simulink model "PID"  (R2025a)
settings: Solver=FixedStepAuto  StartTime=0.0  StopTime=50  FixedStep=0.001  RelTol=1e-3
values from neighbouring files (symbols this model uses):
  g = 9.81    [param.m]
  Iv = diag([1e-2, 8.2e-3, 1.48e-2])    [param.m]
  kd = 0.0487    [param.m]
  Kd_att = [0 0 0]'    [param.m]
  Kd_att_dot = [0.0006 0.0004 0.0]'    [param.m]
  Kd_vel = [0.2 0.2 0]'    [param.m]
  Ki_att = [0 0 0]'    [param.m]
  Ki_att_dot = [0.1 0.1 0.1]'    [param.m]
  Ki_vel = [0.4 0.4 2.0]'    [param.m]
  Kp_att = [6.5 6.5 0.4]'    [param.m]
  Kp_att_dot = [0.053 0.055 0.09]'    [param.m]
  Kp_pos = [0.5 0.5 1]'    [param.m]
  Kp_vel = [1.8 1.8 4]'    [param.m]
  kt = 5.11    [param.m]
  Lpitch = 0.1758    [param.m]
  Lroll = 0.2136    [param.m]
  m = 1.121    [param.m]
settings Model: Creator=huy01  LastModifiedBy=huy01
settings SolverCC: ZeroCrossAlgorithm=Adaptive
settings DebuggingCC: IgnoredZcDiagnostic=none

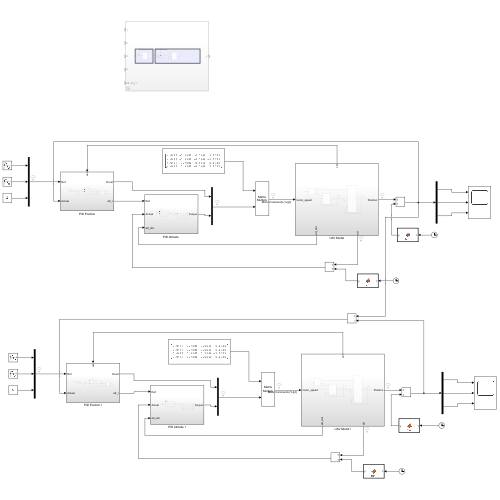
[thumbnail: Simulink's stored preview of the top-level diagram]
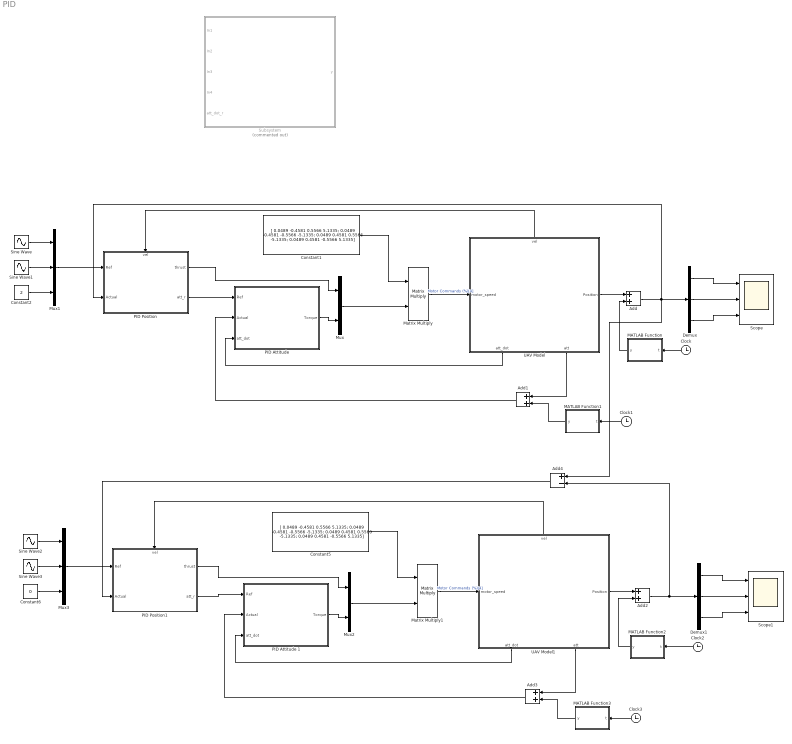
== system PID ==
  Add{,1..3} (4 alike) : Sum
  Add4 : Sum  Inputs=+-
  Clock{,1..3} (4 alike) : Clock
  Constant1 : Constant  Value=|
      | [ 0.0489   -0.4581    0.5566    5.1335;
      |   0.0489   -0.4581   -0.5566   -5.1335;
      |   0.0489    0.4581    0.5566   -5.1335;
      |   0.0489    0.4581   -0.5566    5.1335]
  Constant2 : Constant  Value=2
  Constant5 : Constant  Value=|
      | [ 0.0489   -0.4581    0.5566    5.1335;
      |   0.0489   -0.4581   -0.5566   -5.1335;
      |   0.0489    0.4581    0.5566   -5.1335;
      |   0.0489    0.4581   -0.5566    5.1335]
  Constant6 : Constant  Value=0
  Demux : Demux  Outputs=3
  Demux1 : Demux  Outputs=3
  MATLAB Function : MATLAB Function  TreatAsAtomicUnit=on
  MATLAB Function1 : MATLAB Function  TreatAsAtomicUnit=on
  MATLAB Function2 : MATLAB Function  TreatAsAtomicUnit=on
  MATLAB Function3 : MATLAB Function  TreatAsAtomicUnit=on
  Matrix Multiply : Product  Multiplication=Matrix(*)
  Matrix Multiply1 : Product  Multiplication=Matrix(*)
  Mux : Mux  Inputs=2
  Mux1 : Mux  Inputs=3
  Mux2 : Mux  Inputs=2
  Mux3 : Mux  Inputs=3
  "PID Attitude " : Subsystem
  PID Attitude 1 : Subsystem
  PID Position : Subsystem
      settings: PortSchema="{\"entries\":[{\"content\":{\"sides\":[{\"content\":{\"connectorIds\":[\"In1\",\"In2\"]},\"type\":\"ConnectorPlacement.EquallySpacedRectSide\",\"uuid\":\"8ef4bc25-06d7-445e-a37a-ff1ebe3f11af\"},{\"content\":{\"connectorIds\":[\"Out1\",\"Out2\"],\"side\":\"RIGHT\"},\"type\":\"ConnectorPlacement.EquallySpacedRectSide\",\"uuid\":\"499381c3-f9a0-4f2e-8347-7eacec8f48af\"},{\"content\":{\"connectorIds\":[\"In3\"],\"side\":\"TOP\"},\"type\":\"ConnectorPlacement.EquallySpacedRectSide\",\"uuid\":\"0d907384-0ff5-4165-8e8f-a88dac793d14\"}]},\"type\":\"ConnectorPlacement.EquallySpacedConnector\",\"uuid\":\"f2c7b912-1bff-4caa-903e-36b65c99468e\"}],\"packageUris\":[\"http://schema.mathworks.com/mf0/Connector/R2020b\"],\"version\":\"1.0\"}"
  PID Position1 : Subsystem
      settings: PortSchema="{\"entries\":[{\"content\":{\"sides\":[{\"content\":{\"connectorIds\":[\"In1\",\"In2\"]},\"type\":\"ConnectorPlacement.EquallySpacedRectSide\",\"uuid\":\"757670a2-abb9-46b8-b8ef-ade2779e4005\"},{\"content\":{\"connectorIds\":[\"Out1\",\"Out2\"],\"side\":\"RIGHT\"},\"type\":\"ConnectorPlacement.EquallySpacedRectSide\",\"uuid\":\"80a4837c-f927-466b-93fb-175090a45c5c\"},{\"content\":{\"connectorIds\":[\"In3\"],\"side\":\"TOP\"},\"type\":\"ConnectorPlacement.EquallySpacedRectSide\",\"uuid\":\"6659d1df-ad98-411a-9518-a7cd5dbf3d7b\"}]},\"type\":\"ConnectorPlacement.EquallySpacedConnector\",\"uuid\":\"7846e0cb-a6a7-4697-994f-28587a096689\"}],\"packageUris\":[\"http://schema.mathworks.com/mf0/Connector/R2020b\"],\"version\":\"1.0\"}"
  Scope : Scope  NumInputPorts=3
      settings: ActiveDisplayYMinimum=-0.13419918718369481  ActiveDisplayYMaximum=1.1736814894873611  DataLoggingVariableName=ScopeData2
  Scope1 : Scope  NumInputPorts=3
      settings: ActiveDisplayYMinimum=-2.707243758032325  ActiveDisplayYMaximum=2.7233489767493806  DataLoggingVariableName=ScopeData3
  Sine Wave : Sin  Amplitude=2  Frequency=pi/18  SampleTime=0
  Sine Wave1 : Sin  Amplitude=2  Frequency=pi/18  Phase=pi/2  SampleTime=0
  Sine Wave2 : Sin  Amplitude=4  Frequency=pi/18  SampleTime=0
  Sine Wave3 : Sin  Amplitude=4  Frequency=pi/18  Phase=pi/2  SampleTime=0
  Subsystem : Subsystem  Commented=on
  UAV Model : Subsystem
      settings: PortSchema="{\"entries\":[{\"content\":{\"sides\":[{\"content\":{\"connectorIds\":[\"In1\"]},\"type\":\"ConnectorPlacement.EquallySpacedRectSide\",\"uuid\":\"e9a53653-5fbc-46c1-971d-b6f83c711259\"},{\"content\":{\"connectorIds\":[\"Out1\"],\"side\":\"RIGHT\"},\"type\":\"ConnectorPlacement.EquallySpacedRectSide\",\"uuid\":\"e2104fa5-1b8a-4227-a89f-dda87c76df89\"},{\"content\":{\"connectorIds\":[\"Out4\"],\"side\":\"TOP\"},\"type\":\"ConnectorPlacement.EquallySpacedRectSide\",\"uuid\":\"f4bec026-a14b-467a-8c55-ded87294653f\"},{\"content\":{\"connectorIds\":[\"Out2\",\"Out3\"],\"side\":\"BOTTOM\"},\"type\":\"ConnectorPlacement.EquallySpacedRectSide\",\"uuid\":\"97e6d9ca-da58-485e-9073-412d9dc474d6\"}]},\"type\":\"ConnectorPlacement.EquallySpacedConnector\",\"uuid\":\"03146a94-fd08-496a-b759-aae2d503529b\"}],\"packageUris\":[\"http://schema.mathworks.com/mf0/Connector/R2020b\"],\"version\":\"1.0\"}"
  UAV Model1 : Subsystem
      settings: PortSchema="{\"entries\":[{\"content\":{\"sides\":[{\"content\":{\"connectorIds\":[\"In1\"]},\"type\":\"ConnectorPlacement.EquallySpacedRectSide\",\"uuid\":\"e9a53653-5fbc-46c1-971d-b6f83c711259\"},{\"content\":{\"connectorIds\":[\"Out1\"],\"side\":\"RIGHT\"},\"type\":\"ConnectorPlacement.EquallySpacedRectSide\",\"uuid\":\"e2104fa5-1b8a-4227-a89f-dda87c76df89\"},{\"content\":{\"connectorIds\":[\"Out4\"],\"side\":\"TOP\"},\"type\":\"ConnectorPlacement.EquallySpacedRectSide\",\"uuid\":\"f4bec026-a14b-467a-8c55-ded87294653f\"},{\"content\":{\"connectorIds\":[\"Out2\",\"Out3\"],\"side\":\"BOTTOM\"},\"type\":\"ConnectorPlacement.EquallySpacedRectSide\",\"uuid\":\"97e6d9ca-da58-485e-9073-412d9dc474d6\"}]},\"type\":\"ConnectorPlacement.EquallySpacedConnector\",\"uuid\":\"03146a94-fd08-496a-b759-aae2d503529b\"}],\"packageUris\":[\"http://schema.mathworks.com/mf0/Connector/R2020b\"],\"version\":\"1.0\"}"
  wires:
  PID Position/2(att_r) -> "PID Attitude "/1("Ref ")
  UAV Model/2(att_dot) -> "PID Attitude "/3(att_dot)
  "PID Attitude "/1(Torque) -> Mux/2
  PID Position/1(thrust) -> Mux/1
  Mux/1 -> Matrix Multiply/2
  Constant1/1 -> Matrix Multiply/1
  Mux1/1 -> PID Position/1("Ref ")
  Demux/1 -> Scope/1
  Demux/2 -> Scope/2
  Demux/3 -> Scope/3
  Constant2/1 -> Mux1/3
  Sine Wave/1 -> Mux1/1
  Sine Wave1/1 -> Mux1/2
  MATLAB Function/1(y) -> Add/2
  Clock/1 -> MATLAB Function/1(t)
  UAV Model/1(Position) -> Add/1
  Add/1 -> Add4/1, PID Position/2(Actual), Demux/1
  UAV Model/3(att) -> Add1/1
  Add1/1 -> "PID Attitude "/2(Actual)
  MATLAB Function1/1(y) -> Add1/2
  Clock1/1 -> MATLAB Function1/1(t)
  Matrix Multiply/1 -> UAV Model/1(motor_speed)  "Motor Commands (%)[4]"
  Matrix Multiply1/1 -> UAV Model1/1(motor_speed)  "Motor Commands (%)[4]"
  UAV Model1/1(Position) -> Add2/1
  MATLAB Function2/1(y) -> Add2/2
  MATLAB Function3/1(y) -> Add3/2
  Clock2/1 -> MATLAB Function2/1(t)
  UAV Model1/3(att) -> Add3/1
  Constant6/1 -> Mux3/3
  Sine Wave2/1 -> Mux3/1
  Demux1/3 -> Scope1/3
  PID Position1/2(att_r) -> PID Attitude 1/1("Ref ")
  Constant5/1 -> Matrix Multiply1/1
  Clock3/1 -> MATLAB Function3/1(t)
  Add2/1 -> Demux1/1, Add4/2
  PID Position1/1(thrust) -> Mux2/1
  Mux2/1 -> Matrix Multiply1/2
  UAV Model1/2(att_dot) -> PID Attitude 1/3(att_dot)
  Mux3/1 -> PID Position1/1("Ref ")
  Add3/1 -> PID Attitude 1/2(Actual)
  Demux1/2 -> Scope1/2
  Sine Wave3/1 -> Mux3/2
  PID Attitude 1/1(Torque) -> Mux2/2
  Demux1/1 -> Scope1/1
  Add4/1 -> PID Position1/2(Actual)
  UAV Model/4(vel) -> PID Position/3(vel)
  UAV Model1/4(vel) -> PID Position1/3(vel)

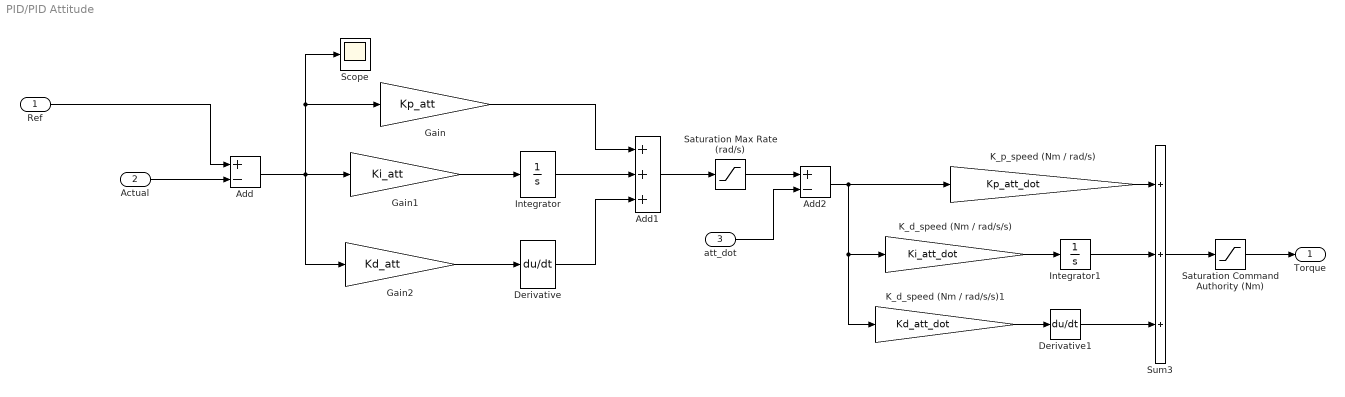
== system PID/PID Attitude  ==
  "Ref " : Inport
  Actual : Inport  Port=2
  att_dot : Inport  Port=3
  Add : Sum  Inputs=+-
  Add1 : Sum  Inputs=+++
  Add2 : Sum  Inputs=+-
  Derivative : Derivative
  Derivative1 : Derivative
  Gain : Gain  Gain=Kp_att
  Gain1 : Gain  Gain=Ki_att
  Gain2 : Gain  Gain=Kd_att
  Integrator : Integrator
  Integrator1 : Integrator
  K_d_speed (Nm / rad/s/s) : Gain  Gain=Ki_att_dot
  K_d_speed (Nm / rad/s/s)1 : Gain  Gain=Kd_att_dot
  K_p_speed (Nm / rad/s) : Gain  Gain=Kp_att_dot
  Saturation Command Authority (Nm) : Saturate  UpperLimit=[1.0915 0.8984 0.0984]'  LowerLimit=-[1.0915 0.8984 0.0984]'
  Saturation Max Rate (rad/s) : Saturate  UpperLimit=10*pi/3*[1 1 1]'  LowerLimit=-10*pi/3*[1 1 1]'
  Scope : Scope
      settings: ActiveDisplayYMinimum=-1  ActiveDisplayYMaximum=1  DataLoggingVariableName=ScopeData5
  Sum3 : Sum  Inputs=+++
  Torque : Outport
  wires:
  Actual/1 -> Add/2
  Add/1 -> Gain2/1, Gain1/1, Gain/1, Scope/1
  Gain1/1 -> Integrator/1
  Integrator/1 -> Add1/2
  Gain/1 -> Add1/1
  Gain2/1 -> Derivative/1
  Derivative/1 -> Add1/3
  "Ref "/1 -> Add/1
  Add1/1 -> Saturation Max Rate (rad/s)/1
  K_d_speed (Nm / rad/s/s)/1 -> Integrator1/1
  K_p_speed (Nm / rad/s)/1 -> Sum3/1
  Saturation Max Rate (rad/s)/1 -> Add2/1
  att_dot/1 -> Add2/2
  Integrator1/1 -> Sum3/2
  K_d_speed (Nm / rad/s/s)1/1 -> Derivative1/1
  Derivative1/1 -> Sum3/3
  Add2/1 -> K_d_speed (Nm / rad/s/s)1/1, K_d_speed (Nm / rad/s/s)/1, K_p_speed (Nm / rad/s)/1
  Sum3/1 -> Saturation Command Authority (Nm)/1
  Saturation Command Authority (Nm)/1 -> Torque/1

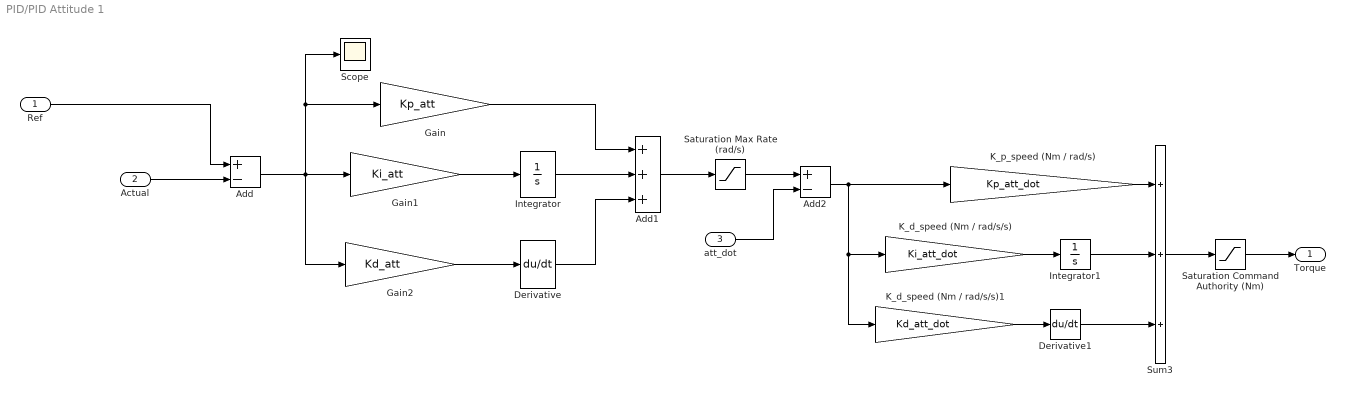
== system PID/PID Attitude 1 ==
  "Ref " : Inport
  Actual : Inport  Port=2
  att_dot : Inport  Port=3
  Add : Sum  Inputs=+-
  Add1 : Sum  Inputs=+++
  Add2 : Sum  Inputs=+-
  Derivative : Derivative
  Derivative1 : Derivative
  Gain : Gain  Gain=Kp_att
  Gain1 : Gain  Gain=Ki_att
  Gain2 : Gain  Gain=Kd_att
  Integrator : Integrator
  Integrator1 : Integrator
  K_d_speed (Nm / rad/s/s) : Gain  Gain=Ki_att_dot
  K_d_speed (Nm / rad/s/s)1 : Gain  Gain=Kd_att_dot
  K_p_speed (Nm / rad/s) : Gain  Gain=Kp_att_dot
  Saturation Command Authority (Nm) : Saturate  UpperLimit=[1.0915 0.8984 0.0984]'  LowerLimit=-[1.0915 0.8984 0.0984]'
  Saturation Max Rate (rad/s) : Saturate  UpperLimit=10*pi/3*[1 1 1]'  LowerLimit=-10*pi/3*[1 1 1]'
  Scope : Scope
      settings: ActiveDisplayYMinimum=-1  ActiveDisplayYMaximum=1  DataLoggingVariableName=ScopeData5
  Sum3 : Sum  Inputs=+++
  Torque : Outport
  wires:
  Actual/1 -> Add/2
  Add/1 -> Gain2/1, Gain1/1, Gain/1, Scope/1
  Gain1/1 -> Integrator/1
  Integrator/1 -> Add1/2
  Gain/1 -> Add1/1
  Gain2/1 -> Derivative/1
  Derivative/1 -> Add1/3
  "Ref "/1 -> Add/1
  Add1/1 -> Saturation Max Rate (rad/s)/1
  K_d_speed (Nm / rad/s/s)/1 -> Integrator1/1
  K_p_speed (Nm / rad/s)/1 -> Sum3/1
  Saturation Max Rate (rad/s)/1 -> Add2/1
  att_dot/1 -> Add2/2
  Integrator1/1 -> Sum3/2
  K_d_speed (Nm / rad/s/s)1/1 -> Derivative1/1
  Derivative1/1 -> Sum3/3
  Add2/1 -> K_d_speed (Nm / rad/s/s)1/1, K_d_speed (Nm / rad/s/s)/1, K_p_speed (Nm / rad/s)/1
  Sum3/1 -> Saturation Command Authority (Nm)/1
  Saturation Command Authority (Nm)/1 -> Torque/1

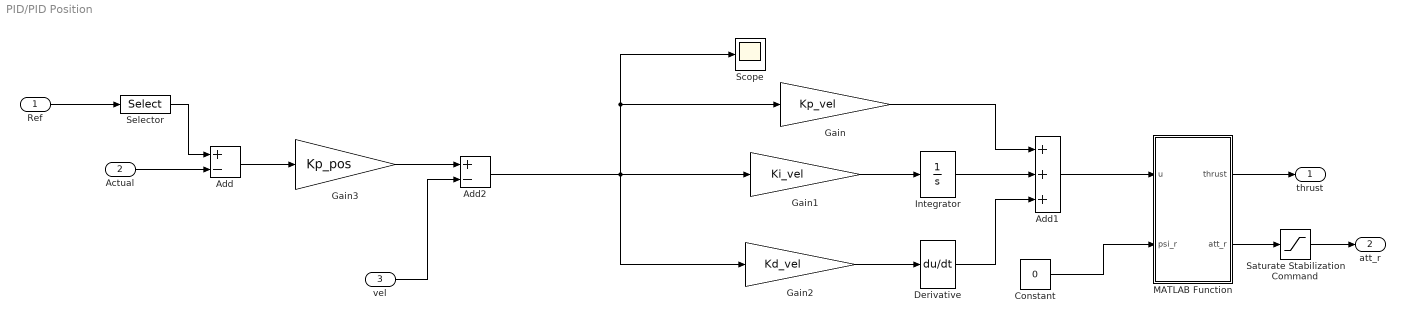
== system PID/PID Position ==
  "Ref " : Inport
  Actual : Inport  Port=2
  vel : Inport  Port=3
  Add : Sum  Inputs=+-
  Add1 : Sum  Inputs=+++
  Add2 : Sum  Inputs=+-
  Constant : Constant  Value=0
  Derivative : Derivative
  Gain : Gain  Gain=Kp_vel
  Gain1 : Gain  Gain=Ki_vel
  Gain2 : Gain  Gain=Kd_vel
  Gain3 : Gain  Gain=Kp_pos
  Integrator : Integrator
  MATLAB Function : MATLAB Function  TreatAsAtomicUnit=on  mask{m=m, g=g}
      mask prompts: m "Mass"; g "Gravity"
  Saturate Stabilization Command : Saturate  UpperLimit=[pi/4 pi/4 inf]'  LowerLimit=[-pi/4 -pi/4 -inf]'
  Scope : Scope
      settings: ActiveDisplayYMinimum=-3.266677596790764  ActiveDisplayYMaximum=4.2877709714359939  DataLoggingVariableName=ScopeData4
  Selector : Selector  InputPortWidth=3  IndexOptions=Index vector (dialog)  Indices=[1:3]  OutputSizes=1
  thrust : Outport
  att_r : Outport  Port=2
  wires:
  Actual/1 -> Add/2
  Gain1/1 -> Integrator/1
  Integrator/1 -> Add1/2
  Gain/1 -> Add1/1
  Gain2/1 -> Derivative/1
  Derivative/1 -> Add1/3
  Add1/1 -> MATLAB Function/1(u)
  "Ref "/1 -> Selector/1
  Selector/1 -> Add/1
  MATLAB Function/1(thrust) -> thrust/1
  MATLAB Function/2(att_r) -> Saturate Stabilization Command/1
  Saturate Stabilization Command/1 -> att_r/1
  Constant/1 -> MATLAB Function/2(psi_r)
  Add/1 -> Gain3/1
  Gain3/1 -> Add2/1
  Add2/1 -> Gain2/1, Gain1/1, Gain/1, Scope/1
  vel/1 -> Add2/2

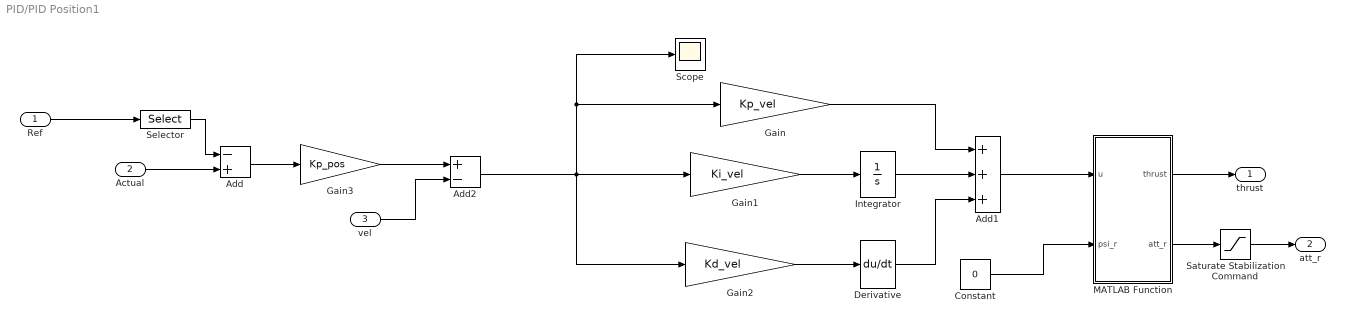
== system PID/PID Position1 ==
  "Ref " : Inport
  Actual : Inport  Port=2
  vel : Inport  Port=3
  Add : Sum  Inputs=-+
  Add1 : Sum  Inputs=+++
  Add2 : Sum  Inputs=+-
  Constant : Constant  Value=0
  Derivative : Derivative
  Gain : Gain  Gain=Kp_vel
  Gain1 : Gain  Gain=Ki_vel
  Gain2 : Gain  Gain=Kd_vel
  Gain3 : Gain  Gain=Kp_pos
  Integrator : Integrator
  MATLAB Function : MATLAB Function  TreatAsAtomicUnit=on  mask{m=m, g=g}
      mask prompts: m "Mass"; g "Gravity"
  Saturate Stabilization Command : Saturate  UpperLimit=[pi/4 pi/4 inf]'  LowerLimit=[-pi/4 -pi/4 -inf]'
  Scope : Scope
      settings: ActiveDisplayYMinimum=-3.266677596790764  ActiveDisplayYMaximum=4.2877709714359939  DataLoggingVariableName=ScopeData4
  Selector : Selector  InputPortWidth=3  IndexOptions=Index vector (dialog)  Indices=[1:3]  OutputSizes=1
  thrust : Outport
  att_r : Outport  Port=2
  wires:
  Actual/1 -> Add/2
  Gain1/1 -> Integrator/1
  Integrator/1 -> Add1/2
  Gain/1 -> Add1/1
  Gain2/1 -> Derivative/1
  Derivative/1 -> Add1/3
  Add1/1 -> MATLAB Function/1(u)
  "Ref "/1 -> Selector/1
  Selector/1 -> Add/1
  MATLAB Function/1(thrust) -> thrust/1
  MATLAB Function/2(att_r) -> Saturate Stabilization Command/1
  Saturate Stabilization Command/1 -> att_r/1
  Constant/1 -> MATLAB Function/2(psi_r)
  Add/1 -> Gain3/1
  Gain3/1 -> Add2/1
  Add2/1 -> Gain2/1, Scope/1, Gain/1, Gain1/1
  vel/1 -> Add2/2

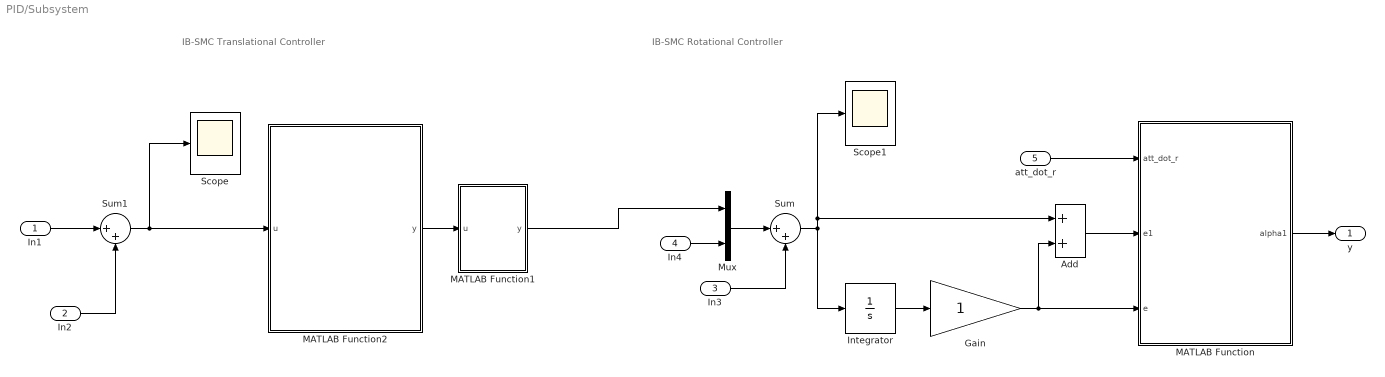
== system PID/Subsystem ==
  note: IB-SMC Translational Controller
  note: IB-SMC Rotational Controller
  In1 : Inport
  In2 : Inport  Port=2
  In3 : Inport  Port=3
  In4 : Inport  Port=4
  att_dot_r : Inport  Port=5
  Add : Sum
  Gain : Gain
  Integrator : Integrator
  MATLAB Function : MATLAB Function  TreatAsAtomicUnit=on
  MATLAB Function1 : MATLAB Function  TreatAsAtomicUnit=on
  MATLAB Function2 : MATLAB Function  TreatAsAtomicUnit=on
  Mux : Mux  Inputs=2
  Scope : Scope
  Scope1 : Scope
  Sum : Sum  Inputs=|++
  Sum1 : Sum  Inputs=|++
  y : Outport
  wires:
  Sum1/1 -> Scope/1, MATLAB Function2/1(u)
  In3/1 -> Sum/2
  MATLAB Function/1(alpha1) -> y/1
  Sum/1 -> Scope1/1, Add/1, Integrator/1
  MATLAB Function2/1(y) -> MATLAB Function1/1(u)
  In2/1 -> Sum1/2
  In1/1 -> Sum1/1
  Mux/1 -> Sum/1
  MATLAB Function1/1(y) -> Mux/1
  In4/1 -> Mux/2
  Integrator/1 -> Gain/1
  Gain/1 -> Add/2, MATLAB Function/3(e)
  Add/1 -> MATLAB Function/2(e1)
  att_dot_r/1 -> MATLAB Function/1(att_dot_r)

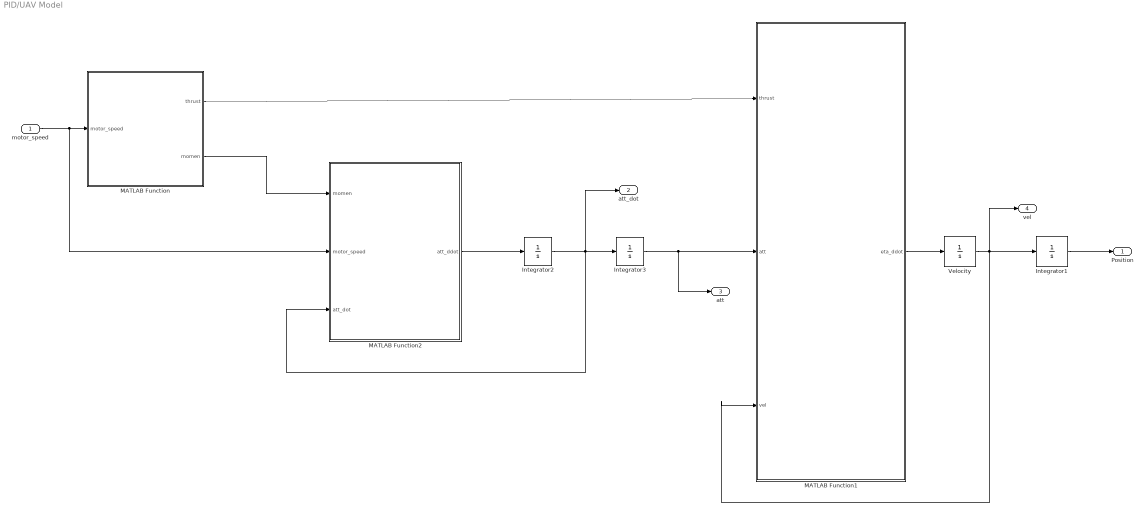
== system PID/UAV Model ==
  motor_speed : Inport
  Integrator1 : Integrator  InitialCondition=[0,0,0]'
  Integrator2 : Integrator  InitialCondition=[0,0,0]'
  Integrator3 : Integrator  InitialCondition=[0,0,0]'
  MATLAB Function : MATLAB Function  TreatAsAtomicUnit=on  mask{kt=kt, kd=kd, d=0, Lroll=Lroll, Lpitch=Lpitch}
      mask prompts: kt "The thrust coefficient (kt)"; kd "The drag force coefficient (kd)"; d "The distance between the center of the mass and the axis of the propeller (d)"
  MATLAB Function1 : MATLAB Function  TreatAsAtomicUnit=on  mask{m=m, k123=zeros(3,1), drag=off, g=g}
      mask prompts: m "The mass of quadrotor"; k123 "Drag force coefficient [3]"; drag "Drag force"; g "Gravity Acceleration"
  MATLAB Function2 : MATLAB Function  TreatAsAtomicUnit=on  mask{gyro_eff=off, aero_friction=off, k456=zeros(3,1), Iv=Iv, Ir=0}
      mask prompts: gyro_eff "Gyroscopic effects"; aero_friction "Aerodynamic Friction"; k456 "Drag force coefficient [3]"; Iv "Iv [3x3]"
  Velocity : Integrator  InitialCondition=[0,0,0]'
  Position : Outport
  att_dot : Outport  Port=2
  att : Outport  Port=3
  vel : Outport  Port=4
  wires:
  Velocity/1 -> vel/1, MATLAB Function1/3(vel), Integrator1/1
  MATLAB Function1/1(eta_ddot) -> Velocity/1
  Integrator3/1 -> att/1, MATLAB Function1/2(att)
  MATLAB Function/2(momen) -> MATLAB Function2/1(momen)
  MATLAB Function/1(thrust) -> MATLAB Function1/1(thrust)
  motor_speed/1 -> MATLAB Function2/2(motor_speed), MATLAB Function/1(motor_speed)
  Integrator1/1 -> Position/1
  MATLAB Function2/1(att_ddot) -> Integrator2/1
  Integrator2/1 -> MATLAB Function2/3(att_dot), att_dot/1, Integrator3/1

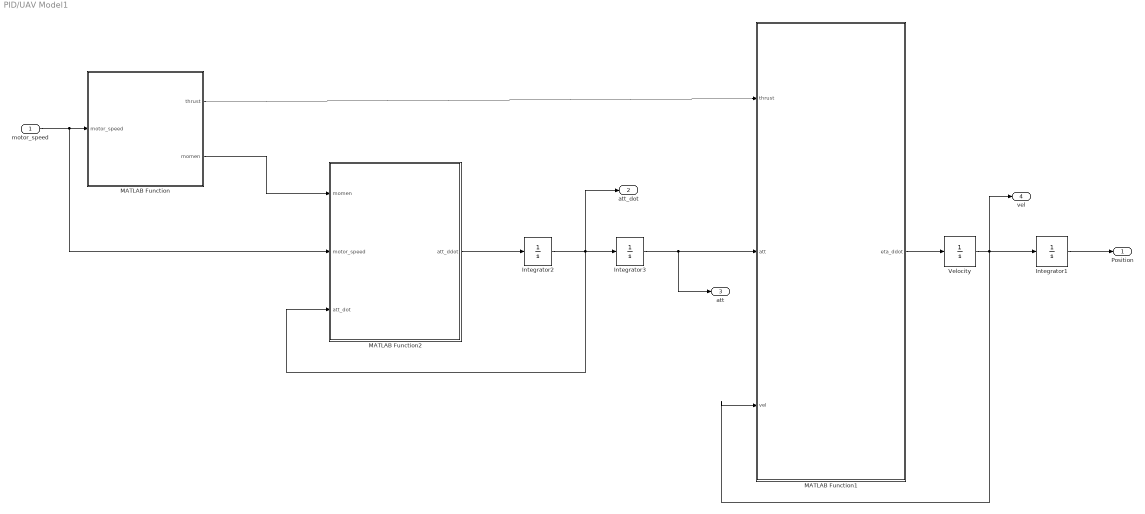
== system PID/UAV Model1 ==
  motor_speed : Inport
  Integrator1 : Integrator  InitialCondition=[0,0,0]'
  Integrator2 : Integrator  InitialCondition=[0,0,0]'
  Integrator3 : Integrator  InitialCondition=[0,0,0]'
  MATLAB Function : MATLAB Function  TreatAsAtomicUnit=on  mask{kt=kt, kd=kd, d=0, Lroll=Lroll, Lpitch=Lpitch}
      mask prompts: kt "The thrust coefficient (kt)"; kd "The drag force coefficient (kd)"; d "The distance between the center of the mass and the axis of the propeller (d)"
  MATLAB Function1 : MATLAB Function  TreatAsAtomicUnit=on  mask{m=m, k123=zeros(3,1), drag=off, g=g}
      mask prompts: m "The mass of quadrotor"; k123 "Drag force coefficient [3]"; drag "Drag force"; g "Gravity Acceleration"
  MATLAB Function2 : MATLAB Function  TreatAsAtomicUnit=on  mask{gyro_eff=off, aero_friction=off, k456=zeros(3,1), Iv=Iv, Ir=0}
      mask prompts: gyro_eff "Gyroscopic effects"; aero_friction "Aerodynamic Friction"; k456 "Drag force coefficient [3]"; Iv "Iv [3x3]"
  Velocity : Integrator  InitialCondition=[0,0,0]'
  Position : Outport
  att_dot : Outport  Port=2
  att : Outport  Port=3
  vel : Outport  Port=4
  wires:
  Velocity/1 -> vel/1, MATLAB Function1/3(vel), Integrator1/1
  MATLAB Function1/1(eta_ddot) -> Velocity/1
  Integrator3/1 -> att/1, MATLAB Function1/2(att)
  MATLAB Function/2(momen) -> MATLAB Function2/1(momen)
  MATLAB Function/1(thrust) -> MATLAB Function1/1(thrust)
  motor_speed/1 -> MATLAB Function2/2(motor_speed), MATLAB Function/1(motor_speed)
  Integrator1/1 -> Position/1
  MATLAB Function2/1(att_ddot) -> Integrator2/1
  Integrator2/1 -> MATLAB Function2/3(att_dot), att_dot/1, Integrator3/1

== matlab function PID/MATLAB Function2 ==
  data: y output; t input
function y = fcn(t)
    
    y = zeros(3,1);

    f = [1 3 7];

    A = 0.0035*sqrt(2/length(f));

    n = 0;

    for k = 1:length(f)
        n = n + A*sin(2*pi*f(k)*t);
    end

    y = n .* [1;1;1];

end

== matlab function PID/MATLAB Function3 ==
  data: y output; t input
function y = fcn(t)
    
    y = zeros(3,1);

    f = [1 3 7 15 30];

    A = 0.0035*sqrt(2/length(f));

    n = 0;

    for k = 1:length(f)
        n = n + A*sin(2*pi*f(k)*t);
    end

    y = n .* [1;1;1];

end

== matlab function PID/PID Position1/MATLAB Function ==
  data: u input; thrust output; psi_r input; att_r output; m parameter; g parameter
function [thrust, att_r] = fcn(u, psi_r, m, g)

    ux = u(1); uy = u(2); uz = u(3);

    thrust = m*sqrt(ux^2 + uy^2 + (uz+g)^2);
    phi_r = asin(m/thrust*(ux*sin(psi_r) - uy*cos(psi_r)));
    theta_r = atan2((ux*cos(psi_r) + uy*sin(psi_r)), (uz+g));

    att_r = [phi_r; theta_r; psi_r];

end

== matlab function PID/UAV Model1/MATLAB Function ==
  data: motor_speed input; thrust output; momen output; d parameter size=1; kt parameter size=1; kd parameter size=1; Lroll parameter; Lpitch parameter
function [thrust, momen] = Translational_Dynamic(motor_speed, d, kt, kd, Lroll, Lpitch)

    thrust = zeros(1,1);
    momen = zeros(3,1);

    input = motor_speed;

    A = [kt, kt, kt, kt;
        -kt*Lroll/2, -kt*Lroll/2, kt*Lroll/2, kt*Lroll/2;
        kt*Lpitch/2, -kt*Lpitch/2, kt*Lpitch/2, -kt*Lpitch/2;
        kd, -kd, -kd, kd];

    output = A*input;

    thrust = output(1);
    momen = output(2:4);

end

== matlab function PID/UAV Model1/MATLAB Function1 ==
  data: thrust input; eta_ddot output; att input; vel input; g parameter; k123 parameter; m parameter; drag parameter
function eta_ddot = Translation_Motion(thrust, att, vel, g, k123, m, drag)

    phi = att(1); theta = att(2); psi = att(3);

    x_dot = vel(1); y_dot = vel(2); z_dot = vel(3);

    k1 = k123(1); k2 = k123(2); k3 = k123(3);

    A = [cos(phi)*sin(theta)*cos(psi) + sin(phi)*sin(psi);
        cos(phi)*sin(theta)*sin(psi) - sin(phi)*cos(psi);
        cos(phi)*cos(theta)];

    d = 1/m .* [k1*x_dot; k2*y_dot; k3*z_dot];

    if drag == 1
        eta_ddot = thrust/m*A - [0, 0, g]' - d;
    else
        eta_ddot = thrust/m*A - [0, 0, g]';
    end
end

== matlab function PID/UAV Model1/MATLAB Function2 ==
  data: momen input; att_ddot output; motor_speed input; att_dot input; gyro_eff parameter; aero_friction parameter; k456 parameter; Iv parameter; Ir parameter
function att_ddot = fcn(momen, motor_speed, att_dot, gyro_eff, aero_friction, k456, Iv, Ir)

    att_ddot = zeros(3,1);

    phi_dot = att_dot(1); theta_dot = att_dot(2); psi_dot = att_dot(3);

    Mx = momen(1); My = momen(2); Mz = momen(3);

    omegaT = motor_speed(4) + motor_speed(3) - motor_speed(2) - motor_speed(1);

    Ix = Iv(1,1); Iy = Iv(2,2); Iz = Iv(3,3);

    k4 = k456(1); k5 = k456(2); k6 = k456(3);

    common_term = [(Iy - Iz)*theta_dot*psi_dot/Ix;
                    (Iz - Ix)*phi_dot*psi_dot/Iy;
                    (Ix - Iy)*phi_dot*theta_dot/Iz] ...
                    + [Mx/Ix; My/Iy; Mz/Iz];

    gyro_term = Ir * [theta_dot/Ix; -phi_dot/Iy; 0] * omegaT;

    drag_term = [k4*phi_dot/Ix;
                k5*theta_dot/Iy;
                k6*psi_dot/Iz];

    if gyro_eff && aero_friction
        att_ddot = common_term - gyro_term - drag_term;
    elseif (~gyro_eff) && aero_friction
        att_ddot = common_term - drag_term;
    elseif gyro_eff && (~aero_friction)
        att_ddot = common_term - gyro_term;
    else 
        att_ddot = common_term;
    end
end

== matlab function PID/UAV Model/MATLAB Function1 ==
  data: thrust input; eta_ddot output; att input; vel input; g parameter; k123 parameter; m parameter; drag parameter
function eta_ddot = Translation_Motion(thrust, att, vel, g, k123, m, drag)

    phi = att(1); theta = att(2); psi = att(3);

    x_dot = vel(1); y_dot = vel(2); z_dot = vel(3);

    k1 = k123(1); k2 = k123(2); k3 = k123(3);

    A = [cos(phi)*sin(theta)*cos(psi) + sin(phi)*sin(psi);
        cos(phi)*sin(theta)*sin(psi) - sin(phi)*cos(psi);
        cos(phi)*cos(theta)];

    d = 1/m .* [k1*x_dot; k2*y_dot; k3*z_dot];

    if drag == 1
        eta_ddot = thrust/m*A - [0, 0, g]' - d;
    else
        eta_ddot = thrust/m*A - [0, 0, g]';
    end
end

== matlab function PID/UAV Model/MATLAB Function ==
  data: motor_speed input; thrust output; momen output; d parameter size=1; kt parameter size=1; kd parameter size=1; Lroll parameter; Lpitch parameter
function [thrust, momen] = Translational_Dynamic(motor_speed, d, kt, kd, Lroll, Lpitch)

    thrust = zeros(1,1);
    momen = zeros(3,1);

    input = motor_speed;

    A = [kt, kt, kt, kt;
        -kt*Lroll/2, -kt*Lroll/2, kt*Lroll/2, kt*Lroll/2;
        kt*Lpitch/2, -kt*Lpitch/2, kt*Lpitch/2, -kt*Lpitch/2;
        kd, -kd, -kd, kd];

    output = A*input;

    thrust = output(1);
    momen = output(2:4);

end

== matlab function PID/UAV Model/MATLAB Function2 ==
  data: momen input; att_ddot output; motor_speed input; att_dot input; gyro_eff parameter; aero_friction parameter; k456 parameter; Iv parameter; Ir parameter
function att_ddot = fcn(momen, motor_speed, att_dot, gyro_eff, aero_friction, k456, Iv, Ir)

    att_ddot = zeros(3,1);

    phi_dot = att_dot(1); theta_dot = att_dot(2); psi_dot = att_dot(3);

    Mx = momen(1); My = momen(2); Mz = momen(3);

    omegaT = motor_speed(4) + motor_speed(3) - motor_speed(2) - motor_speed(1);

    Ix = Iv(1,1); Iy = Iv(2,2); Iz = Iv(3,3);

    k4 = k456(1); k5 = k456(2); k6 = k456(3);

    common_term = [(Iy - Iz)*theta_dot*psi_dot/Ix;
                    (Iz - Ix)*phi_dot*psi_dot/Iy;
                    (Ix - Iy)*phi_dot*theta_dot/Iz] ...
                    + [Mx/Ix; My/Iy; Mz/Iz];

    gyro_term = Ir * [theta_dot/Ix; -phi_dot/Iy; 0] * omegaT;

    drag_term = [k4*phi_dot/Ix;
                k5*theta_dot/Iy;
                k6*psi_dot/Iz];

    if gyro_eff && aero_friction
        att_ddot = common_term - gyro_term - drag_term;
    elseif (~gyro_eff) && aero_friction
        att_ddot = common_term - drag_term;
    elseif gyro_eff && (~aero_friction)
        att_ddot = common_term - gyro_term;
    else 
        att_ddot = common_term;
    end
end

== matlab function PID/Subsystem/MATLAB Function ==
  data: att_dot_r input; alpha1 output; e1 input; e input
function alpha1 = fcn(att_dot_r, e1, e)

    alpha1 = att_dot_r + A1*e1 + e;
end

== matlab function PID/Subsystem/MATLAB Function1 ==
  data: u input; y output
function y = fcn(u)

y = u;

== matlab function PID/Subsystem/MATLAB Function2 ==
  data: u input; y output
function y = fcn(u)

y = u;

== matlab function PID/PID Position/MATLAB Function ==
  data: u input; thrust output; psi_r input; att_r output; m parameter; g parameter
function [thrust, att_r] = fcn(u, psi_r, m, g)

    ux = u(1); uy = u(2); uz = u(3);

    thrust = m*sqrt(ux^2 + uy^2 + (uz+g)^2);
    phi_r = asin(m/thrust*(ux*sin(psi_r) - uy*cos(psi_r)));
    theta_r = atan2((ux*cos(psi_r) + uy*sin(psi_r)), (uz+g));

    att_r = [phi_r; theta_r; psi_r];

end

== matlab function PID/MATLAB Function ==
  data: y output; t input
function y = fcn(t)
    
    y = zeros(3,1);

    f = [1 3 7];

    A = 0.0035*sqrt(2/length(f));

    n = 0;

    for k = 1:length(f)
        n = n + A*sin(2*pi*f(k)*t);
    end

    y = n .* [1;1;1];

end

== matlab function PID/MATLAB Function1 ==
  data: y output; t input
function y = fcn(t)
    
    y = zeros(3,1);

    f = [1 3 7 15 30];

    A = 0.0035*sqrt(2/length(f));

    n = 0;

    for k = 1:length(f)
        n = n + A*sin(2*pi*f(k)*t);
    end

    y = n .* [1;1;1];

end
